simulink model "akvizicija"  (R2015b)
settings: Solver=FixedStepAuto  StartTime=0.0  StopTime=inf  FixedStep=0.001  RelTol=1e-3
undefined symbols (not defined in the file): analoginput
libraries: daqlib x1, arduino_io_lib x1
settings Model: Creator=User  LastModifiedBy=User

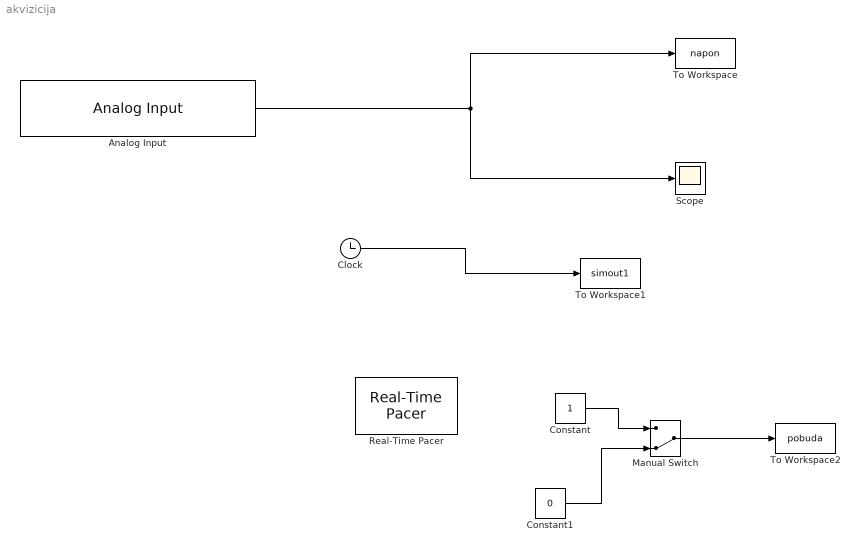
== system akvizicija ==
  Analog Input : daqlib/Analog Input  AcqMode=0  DeviceMenu=mcc 1 (USB-1208FS)  Device=mcc 1 (USB-1208FS)  ObjConstructor=analoginput('mcc',1)  SampleRate=1000  ActualRate=1000  SamplesPerFrame=1  InputType=Differential  NChannelsSelected=1  Channels=1$0$$8$#0$1$$8$#0$2$$8$#0$3$$8$#  NPorts=1 per hardware channel  DataType=double
      settings: SignalType=Sample-based
  Clock : Clock
  Constant : Constant
  Constant1 : Constant  Value=0
  Manual Switch : ManualSwitch  CurrentSetting=0
  Real-Time Pacer : arduino_io_lib/Real-Time Pacer  simTimePerRealTime=1
  Scope : Scope
  To Workspace : ToWorkspace  VariableName=napon  SampleTime=-1
      settings: Save2DSignal=2-D array (concatenate along first dimension)
  To Workspace1 : ToWorkspace  VariableName=simout1  SampleTime=-1
      settings: Save2DSignal=2-D array (concatenate along first dimension)
  To Workspace2 : ToWorkspace  VariableName=pobuda  SampleTime=-1
      settings: Save2DSignal=2-D array (concatenate along first dimension)
  wires:
  Clock/1 -> To Workspace1/1
  Analog Input/1 -> To Workspace/1, Scope/1
  Constant/1 -> Manual Switch/1
  Constant1/1 -> Manual Switch/2
  Manual Switch/1 -> To Workspace2/1
